simulink model "DriverSwRequest_UnitTestHarness2"  (R2026b)
settings: Solver=FixedStepDiscrete  StopTime=2  FixedStep=Ts  EnableMultiTasking=on
undefined symbols (not defined in the file or in its folder): sigbuilder_block, Ts
settings Model: DataDictionary=crs_controllerdic.sldd  Creator=itoy  LastModifiedBy=alexkim
settings DataIOCC: DSMLogging=off  ReturnWorkspaceOutputs=off  SaveFormat=Array  SaveOutput=off  SaveTime=off  SignalLogging=off  VisualizeSimOutput=off
settings OptimizationCC: BlockReduction=off  ConditionallyExecuteInputs=off  DefaultParameterBehavior=Inlined  EfficientTunableParamExpr=on  LifeSpan=Inf  UseDivisionForNetSlopeComputation=on
settings DebuggingCC: AllowSymbolicDim=off  ArithmeticOperatorsInVariantConditions=warning  AssertControl=DisableAll  SFExecutionAtInitializationDiag=none  SFNoUnconditionalDefaultTransitionDiag=warning  SFUnexpectedBacktrackingDiag=warning  SignalInfNanChecking=warning  SolverPrmCheckMsg=warning  StrictBusMsg=ErrorOnBusTreatedAsVector  UniqueDataStoreMsg=warning
settings HardwareCC: ProdEndianess=Unspecified  ProdHWDeviceType=32-bit Generic  ProdLargestAtomicFloat=None
settings ModelReferenceCC: ModelReferenceNumInstancesAllowed=Single  PropagateSignalLabelsOutOfModel=off  PropagateVarSize=Only when enabling
settings SFSimCC: CustomCodeUndefinedFunction=UseInterfaceOnly  SimUseLocalCustomCode=off
settings RTWCC: DLArmComputeVersion=19.05  Description=Embedded Coder  GenCodeOnly=on  GenerateCodeMetricsReport=on  GenerateReport=on  GenerateTraceInfo=on  GenerateTraceReport=on  GenerateTraceReportEml=on  GenerateTraceReportSf=on  GenerateTraceReportSl=on  GenerateWebview=on  IncludeHyperlinkInReport=on  LaunchReport=on  RTWUseLocalCustomCode=off  SystemTargetFile=ert.tlc  TemplateMakefile=ert_default_tmf
settings CodeAppCC: IgnoreCustomStorageClasses=off  StateflowObjectComments=on
settings ERTTargetCC: CastingMode=Standards  DynamicArrayContainerType=coder::array  EnableSignedLeftShifts=off  EnableSignedRightShifts=off  GenerateSampleERTMain=on  GenerateSharedConstants=off  ParenthesesLevel=Maximum  SubcomponentCodeInterfacePackaging=Nonreusable function  SupportNonFinite=off  UtilityFuncGeneration=Shared location
settings ConfigComp: CovExternalEMLEnable=off  CovHTMLOptions=-sRT=1 -sVT=0 -aTS=1 -bRG=1 -bTC=1 -hTR=0 -nFC=0 -nFD=1 -scm=1 -bcm=1 -xEv=0 -xEM=0  CovOutputDir=../reports/slcov_output/$ModelName$  CovSFcnEnable=off  CovSaveCumulativeToWorkspaceVar=on  CovSaveSingleToWorkspaceVar=on  CovScope=ReferencedModels  DVAutomaticStubbing=off  DVDefectChecker=off  DVDetectActiveLogic=on  DVHarnessSource=Signal Editor  DVModelCoverageObjectives=MCDC  DVOutputDir=../reports/sldv_output/$ModelName$  DVSFcnSupport=off  DVSaveReport=on  DVTestSuiteOptimization=Auto

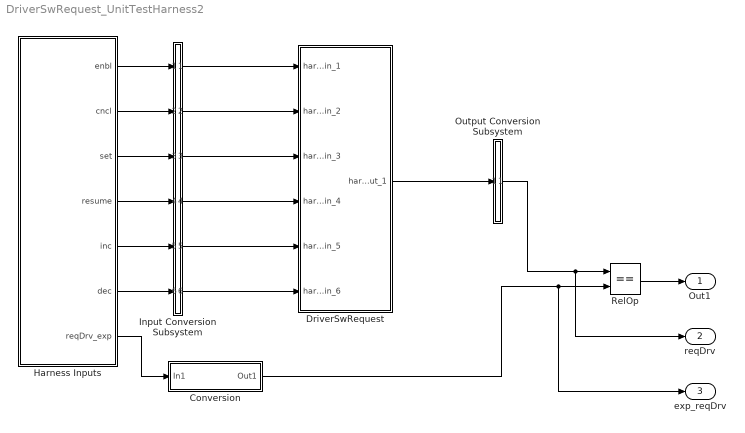
== system DriverSwRequest_UnitTestHarness2 ==
  Conversion : Subsystem
  DriverSwRequest : Subsystem  Tag=__SL_testing_harness_stub_
  Harness Inputs : Subsystem  Tag=STV Subsys  LoadFcn=sigbuilder_block('load');  StartFcn=sigbuilder_block('start');  StopFcn=sigbuilder_block('stop');  ClipboardFcn=sigbuilder_block('clipboard');  mask(Sigbuilder block){tuvar=[0:10]}
      mask init:
      | if ~strcmp(get_param(bdroot(gcb),'SimulationStatus'),'stopped'),tuvar = sigbuilder_block('maskInit'); end
      settings: CopyFcn=sigbuilder_block('copy');  DeleteFcn=sigbuilder_block('delete');  ModelCloseFcn=sigbuilder_block('modelClose');  PreSaveFcn=sigbuilder_block('preSave');  PauseFcn=sigbuilder_block('pause');  ContinueFcn=sigbuilder_block('continue');  NameChangeFcn=sigbuilder_block('namechange');  OpenFcn=sigbuilder_block('open',[1.5 1051.5 541.5 400.5 ]);  CloseFcn=sigbuilder_block('close');
      mask Display: plot(0, 0, 100, 100,[2, 2, 32, 32, 2], [68, 8, 8, 68, 68],[32, 2], [38, 38], [32, 19, 2],[53, 60, 44], [32, 17, 17, 2],[16, 16, 31, 31]);txt = getActiveGroup(gcbh);text(2, 100, txt,'verticalAlignment', 'top');
  Input Conversion Subsystem : Subsystem  Tag=__SLT_ICS__  Description=|
      | Signal spec.
      | and routing
      settings: AttributesFormatString=%<Description>
  Output Conversion Subsystem : Subsystem  Tag=__SLT_OCS__  Description=|
      | Signal spec.
      | and routing
      settings: AttributesFormatString=%<Description>
  RelOp : RelationalOperator  Operator===  OutDataTypeStr=boolean  RndMeth=Simplest  InputSameDT=off
  Out1 : Outport  PortDimensions=[1]  VectorParamsAs1DForOutWhenUnconnected=off
  reqDrv : Outport  Port=2  PortDimensions=[1]  VectorParamsAs1DForOutWhenUnconnected=off
  exp_reqDrv : Outport  Port=3  PortDimensions=[1]  VectorParamsAs1DForOutWhenUnconnected=off
  wires:
  Harness Inputs/1(enbl) -> Input Conversion Subsystem/1(Inport_1)
  Harness Inputs/2(cncl) -> Input Conversion Subsystem/2(Inport_2)
  Harness Inputs/3(set) -> Input Conversion Subsystem/3(Inport_3)
  Harness Inputs/4(resume) -> Input Conversion Subsystem/4(Inport_4)
  Harness Inputs/5(inc) -> Input Conversion Subsystem/5(Inport_5)
  Harness Inputs/6(dec) -> Input Conversion Subsystem/6(Inport_6)
  Output Conversion Subsystem/1(Outport_1) -> reqDrv/1, RelOp/1
  Input Conversion Subsystem/1(Outport_1) -> DriverSwRequest/1(harness_in_1)
  Input Conversion Subsystem/2(Outport_2) -> DriverSwRequest/2(harness_in_2)
  Input Conversion Subsystem/3(Outport_3) -> DriverSwRequest/3(harness_in_3)
  Input Conversion Subsystem/4(Outport_4) -> DriverSwRequest/4(harness_in_4)
  Input Conversion Subsystem/5(Outport_5) -> DriverSwRequest/5(harness_in_5)
  Input Conversion Subsystem/6(Outport_6) -> DriverSwRequest/6(harness_in_6)
  DriverSwRequest/1(harness_out_1) -> Output Conversion Subsystem/1(Inport_1)
  RelOp/1 -> Out1/1
  Harness Inputs/7(reqDrv_exp) -> Conversion/1(In1)
  Conversion/1(Out1) -> exp_reqDrv/1, RelOp/2

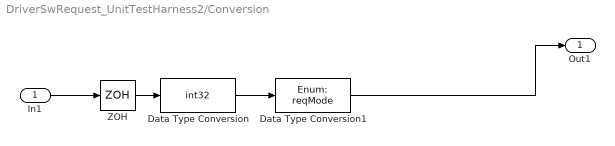
== system DriverSwRequest_UnitTestHarness2/Conversion ==
  In1 : Inport
  Data Type Conversion : DataTypeConversion  OutDataTypeStr=int32  SaturateOnIntegerOverflow=off  RndMeth=Floor
  Data Type Conversion1 : DataTypeConversion  OutDataTypeStr=Enum: reqMode  SaturateOnIntegerOverflow=off  RndMeth=Floor
  ZOH : ZeroOrderHold  SampleTime=Ts
  Out1 : Outport  VectorParamsAs1DForOutWhenUnconnected=off
  wires:
  Data Type Conversion/1 -> Data Type Conversion1/1
  In1/1 -> ZOH/1
  Data Type Conversion1/1 -> Out1/1
  ZOH/1 -> Data Type Conversion/1

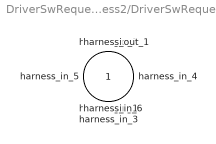
== system DriverSwRequest_UnitTestHarness2/DriverSwRequest ==
  harness_in_1 : Inport
  harness_in_2 : Inport  Port=2
  harness_in_3 : Inport  Port=3
  harness_in_4 : Inport  Port=4
  harness_in_5 : Inport  Port=5
  harness_in_6 : Inport  Port=6
  harness_out_1 : Outport  VectorParamsAs1DForOutWhenUnconnected=off

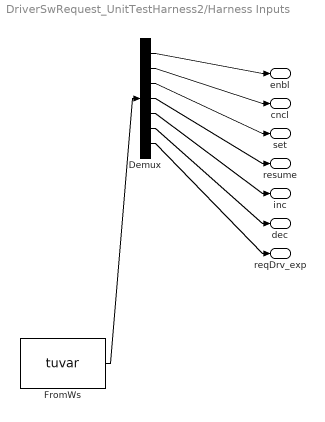
== system DriverSwRequest_UnitTestHarness2/Harness Inputs ==
  Demux : Demux  Tag=STV Demux  Outputs=7
      settings: DisplayOption=none
  FromWs : FromWorkspace  Tag=STV FromWs  VariableName=tuvar  ZeroCross=off  OutputAfterFinalValue=Holding final value
      SigBuilderData=|
      | common.afterFinalStr = 'Hold final value'
      | common.sampleTime = '0'
      | dataSet(1).timeRange = [0 2]
      | dataSet(1).name = 'Enable'
      | dataSet(2).timeRange = [0 2]
      | dataSet(2).name = 'Cancel'
      | dataSet(3).timeRange = [0 2]
      | dataSet(3).name = 'Set'
      | dataSet(4).timeRange = [0 2]
      | dataSet(4).name = 'Resume'
      | dataSet(5).timeRange = [0 2]
      | dataSet(5).name = 'ShortInc'
      | dataSet(6).timeRange = [0 3]
      | dataSet(6).name = 'LongInc'
      | dataSet(7).timeRange = [0 2]
      | dataSet(7).name = 'ShortDec'
      | dataSet(8).timeRange = [0 3]
      | dataSet(8).name = 'LongDec'
      | sbobj.Name = 'Signal Builder'
      | sbobj.Groups(1).Name = 'Enable'
      | sbobj.Groups(1).Signals(1).Name = 'enbl'
      | sbobj.Groups(1).Signals(1).XData = [0 1 1 1.01 1.01 2]
      | sbobj.Groups(1).Signals(1).YData = [0 0 1 1 0 0]
      | sbobj.Groups(1).Signals(2).Name = 'cncl'
      | sbobj.Groups(1).Signals(2).XData = [0 1 1.01 2]
      | sbobj.Groups(1).Signals(2).YData = [0 0 0 0]
      | sbobj.Groups(1).Signals(3).Name = 'set'
      | sbobj.Groups(1).Signals(3).XData = [0 1 1.01 2]
      | sbobj.Groups(1).Signals(3).YData = [0 0 0 0]
      | sbobj.Groups(1).Signals(4).Name = 'resume'
      | sbobj.Groups(1).Signals(4).XData = [0 1 1.01 2]
      | sbobj.Groups(1).Signals(4).YData = [0 0 0 0]
      | sbobj.Groups(1).Signals(5).Name = 'inc'
      | sbobj.Groups(1).Signals(5).XData = [0 1 1.01 2]
      | sbobj.Groups(1).Signals(5).YData = [0 0 0 0]
      | sbobj.Groups(1).Signals(6).Name = 'dec'
      | sbobj.Groups(1).Signals(6).XData = [0 1 1.01 2]
      | sbobj.Groups(1).Signals(6).YData = [0 0 0 0]
      | sbobj.Groups(1).Signals(7).Name = 'reqDrv_exp'
      | sbobj.Groups(1).Signals(7).XData = [0 1 1 1.01 1.01 2]
      | sbobj.Groups(1).Signals(7).YData = [0 0 2 2 0 0]
      | sbobj.Groups(1).TimeRange = [0 2]
      | sbobj.Groups(2).Name = 'Cancel'
      | sbobj.Groups(2).Signals(1).Name = 'enbl'
      | sbobj.Groups(2).Signals(1).XData = [0 1 1.01 2]
      | sbobj.Groups(2).Signals(1).YData = [0 0 0 0]
      | sbobj.Groups(2).Signals(2).Name = 'cncl'
      | sbobj.Groups(2).Signals(2).XData = [0 1 1 1.01 1.01 2]
      | sbobj.Groups(2).Signals(2).YData = [0 0 1 1 0 0]
      | sbobj.Groups(2).Signals(3).Name = 'set'
      | sbobj.Groups(2).Signals(3).XData = [0 1 1.01 2]
      | sbobj.Groups(2).Signals(3).YData = [0 0 0 0]
      | sbobj.Groups(2).Signals(4).Name = 'resume'
      | sbobj.Groups(2).Signals(4).XData = [0 1 1.01 2]
      | sbobj.Groups(2).Signals(4).YData = [0 0 0 0]
      | sbobj.Groups(2).Signals(5).Name = 'inc'
      | sbobj.Groups(2).Signals(5).XData = [0 1 1.01 2]
      | sbobj.Groups(2).Signals(5).YData = [0 0 0 0]
      | sbobj.Groups(2).Signals(6).Name = 'dec'
      | sbobj.Groups(2).Signals(6).XData = [0 1 1.01 2]
      | sbobj.Groups(2).Signals(6).YData = [0 0 0 0]
      | sbobj.Groups(2).Signals(7).Name = 'reqDrv_exp'
      | sbobj.Groups(2).Signals(7).XData = [0 1 1 1.02 1.02 2]
      | sbobj.Groups(2).Signals(7).YData = [0 0 1 1 0 0]
      | sbobj.Groups(2).TimeRange = [0 2]
      | sbobj.Groups(3).Name = 'Set'
      | sbobj.Groups(3).Signals(1).Name = 'enbl'
      | sbobj.Groups(3).Signals(1).XData = [0 1 1 1.01 1.01 2]
      | sbobj.Groups(3).Signals(1).YData = [0 0 0 0 0 0]
      | sbobj.Groups(3).Signals(2).Name = 'cncl'
      | sbobj.Groups(3).Signals(2).XData = [0 1 1 1.01 1.01 2]
      | sbobj.Groups(3).Signals(2).YData = [0 0 0 0 0 0]
      | sbobj.Groups(3).Signals(3).Name = 'set'
      | sbobj.Groups(3).Signals(3).XData = [0 1 1 1.01 1.01 2]
      | sbobj.Groups(3).Signals(3).YData = [0 0 1 1 0 0]
      | sbobj.Groups(3).Signals(4).Name = 'resume'
      | sbobj.Groups(3).Signals(4).XData = [0 1 1 1.01 1.01 2]
      | sbobj.Groups(3).Signals(4).YData = [0 0 0 0 0 0]
      | sbobj.Groups(3).Signals(5).Name = 'inc'
      | sbobj.Groups(3).Signals(5).XData = [0 1 1 1.01 1.01 2]
      | sbobj.Groups(3).Signals(5).YData = [0 0 0 0 0 0]
      | sbobj.Groups(3).Signals(6).Name = 'dec'
      | sbobj.Groups(3).Signals(6).XData = [0 1 1 1.01 1.01 2]
      | sbobj.Groups(3).Signals(6).YData = [0 0 0 0 0 0]
      | sbobj.Groups(3).Signals(7).Name = 'reqDrv_exp'
      | sbobj.Groups(3).Signals(7).XData = [0 1 1 1.01 1.01 2]
      | sbobj.Groups(3).Signals(7).YData = [0 0 3 3 0 0]
      | sbobj.Groups(3).TimeRange = [0 2]
      | sbobj.Groups(4).Name = 'Resume'
      | sbobj.Groups(4).Signals(1).Name = 'enbl'
      | sbobj.Groups(4).Signals(1).XData = [0 1 1 1.01 1.01 2]
      | sbobj.Groups(4).Signals(1).YData = [0 0 0 0 0 0]
      | sbobj.Groups(4).Signals(2).Name = 'cncl'
      | sbobj.Groups(4).Signals(2).XData = [0 1 1 1.01 1.01 2]
      | sbobj.Groups(4).Signals(2).YData = [0 0 0 0 0 0]
      | sbobj.Groups(4).Signals(3).Name = 'set'
      | sbobj.Groups(4).Signals(3).XData = [0 1 1 1.01 1.01 2]
      | sbobj.Groups(4).Signals(3).YData = [0 0 0 0 0 0]
      | sbobj.Groups(4).Signals(4).Name = 'resume'
      | sbobj.Groups(4).Signals(4).XData = [0 1 1 1.01 1.01 2]
      | sbobj.Groups(4).Signals(4).YData = [0 0 1 1 0 0]
      | sbobj.Groups(4).Signals(5).Name = 'inc'
      | sbobj.Groups(4).Signals(5).XData = [0 1 1 1.01 1.01 2]
      | sbobj.Groups(4).Signals(5).YData = [0 0 0 0 0 0]
      | sbobj.Groups(4).Signals(6).Name = 'dec'
      | sbobj.Groups(4).Signals(6).XData = [0 1 1 1.01 1.01 2]
      | sbobj.Groups(4).Signals(6).YData = [0 0 0 0 0 0]
      | sbobj.Groups(4).Signals(7).Name = 'reqDrv_exp'
      | sbobj.Groups(4).Signals(7).XData = [0 1 1 1.01 1.01 2]
      | sbobj.Groups(4).Signals(7).YData = [0 0 4 4 0 0]
      | sbobj.Groups(4).TimeRange = [0 2]
      | sbobj.Groups(5).Name = 'ShortInc'
      | sbobj.Groups(5).Signals(1).Name = 'enbl'
      | sbobj.Groups(5).Signals(1).XData = [0 1 1 1.01 1.01 2]
      | sbobj.Groups(5).Signals(1).YData = [0 0 0 0 0 0]
      | sbobj.Groups(5).Signals(2).Name = 'cncl'
      | sbobj.Groups(5).Signals(2).XData = [0 1 1 1.01 1.01 2]
      | sbobj.Groups(5).Signals(2).YData = [0 0 0 0 0 0]
      | sbobj.Groups(5).Signals(3).Name = 'set'
      | sbobj.Groups(5).Signals(3).XData = [0 1 1 1.01 1.01 2]
      | sbobj.Groups(5).Signals(3).YData = [0 0 0 0 0 0]
      | sbobj.Groups(5).Signals(4).Name = 'resume'
      | sbobj.Groups(5).Signals(4).XData = [0 1 1 1.01 1.01 2]
      | sbobj.Groups(5).Signals(4).YData = [0 0 0 0 0 0]
      | sbobj.Groups(5).Signals(5).Name = 'inc'
      | sbobj.Groups(5).Signals(5).XData = [0 1 1 1.01 1.01 2]
      | sbobj.Groups(5).Signals(5).YData = [0 0 1 1 0 0]
      | sbobj.Groups(5).Signals(6).Name = 'dec'
      | sbobj.Groups(5).Signals(6).XData = [0 1 1 1.01 1.01 2]
      | sbobj.Groups(5).Signals(6).YData = [0 0 0 0 0 0]
      | sbobj.Groups(5).Signals(7).Name = 'reqDrv_exp'
      | sbobj.Groups(5).Signals(7).XData = [0 1 1 1.01 1.01 2]
      | sbobj.Groups(5).Signals(7).YData = [0 0 5 5 0 0]
      | sbobj.Groups(5).TimeRange = [0 2]
      | sbobj.Groups(6).Name = 'LongInc'
      | sbobj.Groups(6).Signals(1).Name = 'enbl'
      | sbobj.Groups(6).Signals(1).XData = [0 1 1 1.01 1.01 1.02 1.5 1.5 2 2 3]
      | sbobj.Groups(6).Signals(1).YData = [0 0 0 0 0 0 0 0 0 0 0]
      | sbobj.Groups(6).Signals(2).Name = 'cncl'
      | sbobj.Groups(6).Signals(2).XData = [0 1 1 1.01 1.01 1.02 1.5 1.5 2 2 3]
      | sbobj.Groups(6).Signals(2).YData = [0 0 0 0 0 0 0 0 0 0 0]
      | sbobj.Groups(6).Signals(3).Name = 'set'
      | sbobj.Groups(6).Signals(3).XData = [0 1 1 1.01 1.01 1.02 1.5 1.5 2 2 3]
      | sbobj.Groups(6).Signals(3).YData = [0 0 0 0 0 0 0 0 0 0 0]
      | sbobj.Groups(6).Signals(4).Name = 'resume'
      | sbobj.Groups(6).Signals(4).XData = [0 1 1 1.01 1.01 1.02 1.5 1.5 2 2 3]
      | sbobj.Groups(6).Signals(4).YData = [0 0 0 0 0 0 0 0 0 0 0]
      | sbobj.Groups(6).Signals(5).Name = 'inc'
      | sbobj.Groups(6).Signals(5).XData = [0 1 1 1.01 1.01 1.02 1.5 1.5 2 2 3]
      | sbobj.Groups(6).Signals(5).YData = [0 0 1 1 1 1 1 1 1 0 0]
      | sbobj.Groups(6).Signals(6).Name = 'dec'
      | sbobj.Groups(6).Signals(6).XData = [0 1 1 1.01 1.01 1.02 1.5 1.5 2 2 3]
      | sbobj.Groups(6).Signals(6).YData = [0 0 0 0 0 0 0 0 0 0 0]
      | sbobj.Groups(6).Signals(7).Name = 'reqDrv_exp'
      | sbobj.Groups(6).Signals(7).XData = [0 1 1 1.01 1.01 1.02 1.5 1.5 2 2 3]
      | sbobj.Groups(6).Signals(7).YData = [0 0 5 5 6 6 6 7 7 0 0]
      | sbobj.Groups(6).TimeRange = [0 3]
      | sbobj.Groups(7).Name = 'ShortDec'
      | sbobj.Groups(7).Signals(1).Name = 'enbl'
      | sbobj.Groups(7).Signals(1).XData = [0 1 1 1.01 1.01 2]
      | sbobj.Groups(7).Signals(1).YData = [0 0 0 0 0 0]
      | sbobj.Groups(7).Signals(2).Name = 'cncl'
      | sbobj.Groups(7).Signals(2).XData = [0 1 1 1.01 1.01 2]
      | sbobj.Groups(7).Signals(2).YData = [0 0 0 0 0 0]
      | sbobj.Groups(7).Signals(3).Name = 'set'
      | sbobj.Groups(7).Signals(3).XData = [0 1 1 1.01 1.01 2]
      | sbobj.Groups(7).Signals(3).YData = [0 0 0 0 0 0]
      | sbobj.Groups(7).Signals(4).Name = 'resume'
      | sbobj.Groups(7).Signals(4).XData = [0 1 1 1.01 1.01 2]
      | sbobj.Groups(7).Signals(4).YData = [0 0 0 0 0 0]
      | sbobj.Groups(7).Signals(5).Name = 'inc'
      | sbobj.Groups(7).Signals(5).XData = [0 1 1 1.01 1.01 2]
      | sbobj.Groups(7).Signals(5).YData = [0 0 0 0 0 0]
      | sbobj.Groups(7).Signals(6).Name = 'dec'
      | sbobj.Groups(7).Signals(6).XData = [0 1 1 1.01 1.01 2]
      | sbobj.Groups(7).Signals(6).YData = [0 0 1 1 0 0]
      | sbobj.Groups(7).Signals(7).Name = 'reqDrv_exp'
      | sbobj.Groups(7).Signals(7).XData = [0 1 1 1.01 1.01 2]
      | sbobj.Groups(7).Signals(7).YData = [0 0 8 8 0 0]
      | sbobj.Groups(7).TimeRange = [0 2]
      | sbobj.Groups(8).Name = 'LongDec'
      | sbobj.Groups(8).Signals(1).Name = 'enbl'
      | sbobj.Groups(8).Signals(1).XData = [0 1 1 1.01 1.01 1.02 1.5 1.5 2 2 3]
      | sbobj.Groups(8).Signals(1).YData = [0 0 0 0 0 0 0 0 0 0 0]
      | sbobj.Groups(8).Signals(2).Name = 'cncl'
      | sbobj.Groups(8).Signals(2).XData = [0 1 1 1.01 1.01 1.02 1.5 1.5 2 2 3]
      | sbobj.Groups(8).Signals(2).YData = [0 0 0 0 0 0 0 0 0 0 0]
      | sbobj.Groups(8).Signals(3).Name = 'set'
      | sbobj.Groups(8).Signals(3).XData = [0 1 1 1.01 1.01 1.02 1.5 1.5 2 2 3]
      | sbobj.Groups(8).Signals(3).YData = [0 0 0 0 0 0 0 0 0 0 0]
      | sbobj.Groups(8).Signals(4).Name = 'resume'
      | sbobj.Groups(8).Signals(4).XData = [0 1 1 1.01 1.01 1.02 1.5 1.5 2 2 3]
      | sbobj.Groups(8).Signals(4).YData = [0 0 0 0 0 0 0 0 0 0 0]
      | sbobj.Groups(8).Signals(5).Name = 'inc'
      | sbobj.Groups(8).Signals(5).XData = [0 1 1 1.01 1.01 1.02 1.5 1.5 2 2 3]
      | sbobj.Groups(8).Signals(5).YData = [0 0 0 0 0 0 0 0 0 0 0]
      | sbobj.Groups(8).Signals(6).Name = 'dec'
      | sbobj.Groups(8).Signals(6).XData = [0 1 1 1.01 1.01 1.02 1.5 1.5 2 2 3]
      | sbobj.Groups(8).Signals(6).YData = [0 0 1 1 1 1 1 1 1 0 0]
      | sbobj.Groups(8).Signals(7).Name = 'reqDrv_exp'
      | sbobj.Groups(8).Signals(7).XData = [0 1 1 1.01 1.01 1.02 1.5 1.5 2 2 3]
      | sbobj.Groups(8).Signals(7).YData = [0 0 8 8 9 9 9 10 10 0 0]
      | sbobj.Groups(8).TimeRange = [0 3]
  enbl : Outport  Tag=STV Outport  VectorParamsAs1DForOutWhenUnconnected=off
  cncl : Outport  Tag=STV Outport  Port=2  VectorParamsAs1DForOutWhenUnconnected=off
  set : Outport  Tag=STV Outport  Port=3  VectorParamsAs1DForOutWhenUnconnected=off
  resume : Outport  Tag=STV Outport  Port=4  VectorParamsAs1DForOutWhenUnconnected=off
  inc : Outport  Tag=STV Outport  Port=5  VectorParamsAs1DForOutWhenUnconnected=off
  dec : Outport  Tag=STV Outport  Port=6  VectorParamsAs1DForOutWhenUnconnected=off
  reqDrv_exp : Outport  Tag=STV Outport  Port=7  VectorParamsAs1DForOutWhenUnconnected=off
  wires:
  FromWs/1 -> Demux/1
  Demux/1 -> enbl/1
  Demux/2 -> cncl/1
  Demux/3 -> set/1
  Demux/4 -> resume/1
  Demux/5 -> inc/1
  Demux/6 -> dec/1
  Demux/7 -> reqDrv_exp/1

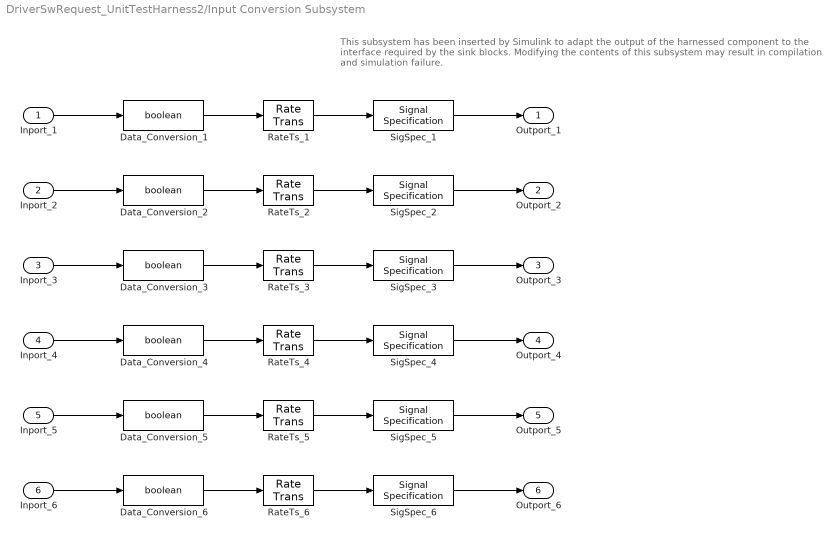
== system DriverSwRequest_UnitTestHarness2/Input Conversion Subsystem ==
  note: This subsystem has been inserted by Simulink to adapt the output of the harnessed component to the interface required by the sink blocks.
      |  Modifying the contents of this subsystem may result in compilation and simulation failure.
  Inport_1 : Inport
  Inport_2 : Inport  Port=2
  Inport_3 : Inport  Port=3
  Inport_4 : Inport  Port=4
  Inport_5 : Inport  Port=5
  Inport_6 : Inport  Port=6
  Data_Conversion_{1..6} (6 alike) : DataTypeConversion  OutDataTypeStr=boolean
  RateTs_{1..6} (6 alike) : RateTransition  OutPortSampleTime=0.01
  SigSpec_{1..6} (6 alike) : SignalSpecification  OutDataTypeStr=boolean  Dimensions=[1]  SampleTime=0.01
  Outport_1 : Outport  VectorParamsAs1DForOutWhenUnconnected=off
  Outport_2 : Outport  Port=2  VectorParamsAs1DForOutWhenUnconnected=off
  Outport_3 : Outport  Port=3  VectorParamsAs1DForOutWhenUnconnected=off
  Outport_4 : Outport  Port=4  VectorParamsAs1DForOutWhenUnconnected=off
  Outport_5 : Outport  Port=5  VectorParamsAs1DForOutWhenUnconnected=off
  Outport_6 : Outport  Port=6  VectorParamsAs1DForOutWhenUnconnected=off
  wires:
  SigSpec_1/1 -> Outport_1/1
  RateTs_1/1 -> SigSpec_1/1
  Data_Conversion_1/1 -> RateTs_1/1
  Inport_1/1 -> Data_Conversion_1/1
  SigSpec_2/1 -> Outport_2/1
  RateTs_2/1 -> SigSpec_2/1
  Data_Conversion_2/1 -> RateTs_2/1
  Inport_2/1 -> Data_Conversion_2/1
  SigSpec_3/1 -> Outport_3/1
  RateTs_3/1 -> SigSpec_3/1
  Data_Conversion_3/1 -> RateTs_3/1
  Inport_3/1 -> Data_Conversion_3/1
  SigSpec_4/1 -> Outport_4/1
  RateTs_4/1 -> SigSpec_4/1
  Data_Conversion_4/1 -> RateTs_4/1
  Inport_4/1 -> Data_Conversion_4/1
  SigSpec_5/1 -> Outport_5/1
  RateTs_5/1 -> SigSpec_5/1
  Data_Conversion_5/1 -> RateTs_5/1
  Inport_5/1 -> Data_Conversion_5/1
  SigSpec_6/1 -> Outport_6/1
  RateTs_6/1 -> SigSpec_6/1
  Data_Conversion_6/1 -> RateTs_6/1
  Inport_6/1 -> Data_Conversion_6/1

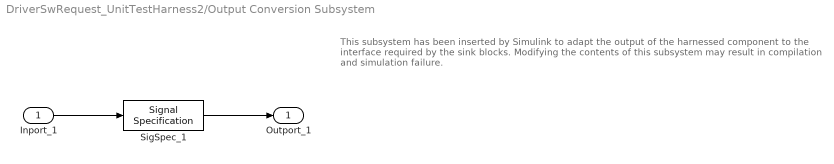
== system DriverSwRequest_UnitTestHarness2/Output Conversion Subsystem ==
  note: This subsystem has been inserted by Simulink to adapt the output of the harnessed component to the interface required by the sink blocks.
      |  Modifying the contents of this subsystem may result in compilation and simulation failure.
  Inport_1 : Inport
  SigSpec_1 : SignalSpecification  OutDataTypeStr=Enum: reqMode  Dimensions=[1]  SampleTime=0.01
  Outport_1 : Outport  VectorParamsAs1DForOutWhenUnconnected=off
  wires:
  Inport_1/1 -> SigSpec_1/1
  SigSpec_1/1 -> Outport_1/1
